simulink library "SHCLib"  (R2023a)
settings: Solver=VariableStepAuto  StartTime=0.0  StopTime=10.0  RelTol=1e-3
settings Model: Creator=hwx20  LastModifiedBy=hwx20

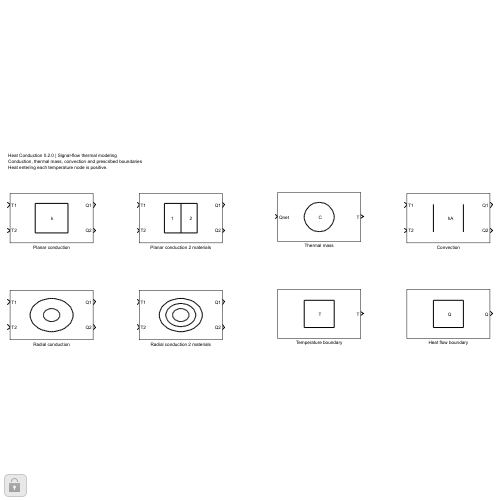
[thumbnail: Simulink's stored preview of the top-level diagram]
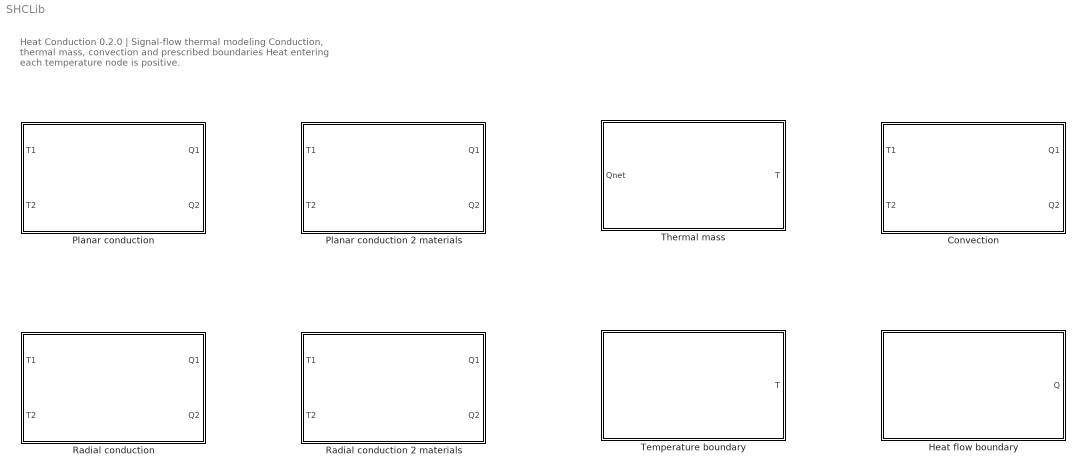
== system SHCLib ==
  note: Heat Conduction 0.2.0 | Signal-flow thermal modeling
      | Conduction, thermal mass, convection and prescribed boundaries
      | Heat entering each temperature node is positive.
  Convection : Subsystem  mask(SHC Convection){h=10, area=0.5}
      mask prompts: h "Heat transfer coefficient / 对流换热系数 [W/(m^2 K)]"; area "Heat transfer area / 换热面积 [m^2]"
      mask help:
      | Constant-coefficient convection / 常系数对流换热.
      | Inputs T1,T2 [same temperature scale]; outputs Q1,Q2 [W].
      | Q1=h*area*(T2-T1), Q2=-Q1. Positive heat enters the corresponding node.
      | h=0 gives zero heat flow. This element has no thermal storage.
      | It does not calculate fluid flow or infer h from flow conditions.
      mask init:
      | validateattributes(area,{'numeric'},{'real','scalar','finite','positive'},'SHC','area');
      | validateattributes(h,{'numeric'},{'real','scalar','finite','nonnegative'},'SHC','h');
      | validateattributes(h*area,{'numeric'},{'real','scalar','finite','nonnegative'},'SHC','convective conductance');
      mask Help: disp(get_param(gcb,'MaskDescription'));
      mask Display:
      | plot([.32 .32],[.22 .78]);
      | plot([.68 .68],[.22 .78]);
      | text(.5,.5,'hA');
      | port_label('input',1,'T1');
      | port_label('input',2,'T2');
      | port_label('output',1,'Q1');
      | port_label('output',2,'Q2');
  Heat flow boundary : Subsystem  mask(SHC Heat flow boundary){power=100}
      mask prompts: power "Prescribed heat power / 规定热功率 [W]"
      mask help:
      | Constant prescribed heat power / 恒热功率边界.
      | Output Q [W]: positive adds heat; negative removes heat.
      | Add this signal to the receiving thermal mass net heat input.
      | This is total heat power, not area-specific heat flux [W/m^2].
      | Use a standard Simulink source for a time-dependent heat-power signal.
      mask init:
      | validateattributes(power,{'numeric'},{'real','scalar','finite'},'SHC','power');
      mask Help: disp(get_param(gcb,'MaskDescription'));
      mask Display:
      | plot([.32 .32 .68 .68 .32],[.22 .78 .78 .22 .22]);
      | text(.5,.5,'Q');
      | port_label('output',1,'Q');
  Planar conduction : Subsystem  mask(SHC Planar conduction){lambda=10, distance=0.01, area=0.02}
      mask prompts: lambda "Thermal conductivity / 导热系数 [W/(m K)]"; distance "Distance between temperature nodes / 节点间距离 [m]"; area "Heat transfer area / 传热面积 [m^2]"
      mask help:
      | Single-material planar conduction.
      | R=distance/(lambda*area).
      | T1/T2: temperature [degC or K, use the same scale].
      | Q1/Q2: heat entering node 1/node 2 [W].
      | Q1=(T2-T1)/R; Q2=-Q1.
      | This is a resistance element. Add external thermal capacitances for storage.
      mask init:
      | validateattributes(lambda,{'numeric'},{'real','scalar','finite','positive'},'SHC','lambda');
      | validateattributes(distance,{'numeric'},{'real','scalar','finite','positive'},'SHC','distance');
      | validateattributes(area,{'numeric'},{'real','scalar','finite','positive'},'SHC','area');
      | 
      | validateattributes(distance/(lambda*area),{'numeric'},{'real','scalar','finite','positive'},'SHC','R_total');
      mask Help: disp(get_param(gcb,'MaskDescription'));
      mask Display:
      | plot([.30 .30 .70 .70 .30],[.20 .80 .80 .20 .20]);
      | text(.50,.50,'k');
      | port_label('input',1,'T1');
      | port_label('input',2,'T2');
      | port_label('output',1,'Q1');
      | port_label('output',2,'Q2');
  Planar conduction 2 materials : Subsystem  mask(SHC Planar conduction 2 materials){lambda1=1, distance1=0.005, lambda2=2, distance2=0.002, area=0.01, ctr=0.2}
      mask prompts: lambda1 "Material 1 conductivity / 材料1导热系数 [W/(m K)]"; distance1 "Node 1 to interface / 节点1到界面距离 [m]"; lambda2 "Material 2 conductivity / 材料2导热系数 [W/(m K)]"; distance2 "Interface to node 2 / 界面到节点2距离 [m]"; area "Heat transfer area / 传热面积 [m^2]"; ctr "Total contact resistance / 界面总热阻 [K/W]"
      mask help:
      | Two planar material layers in series, with optional contact resistance.
      | R=distance1/(lambda1*area)+distance2/(lambda2*area)+ctr.
      | ctr is TOTAL resistance [K/W], not area-specific resistance.
      | T1/T2: temperature [degC or K, use the same scale].
      | Q1/Q2: heat entering node 1/node 2 [W].
      | Q1=(T2-T1)/R; Q2=-Q1.
      | This is a resistance element. Add external thermal capacitances for storage.
      mask init:
      | validateattributes(lambda1,{'numeric'},{'real','scalar','finite','positive'},'SHC','lambda1');
      | validateattributes(lambda2,{'numeric'},{'real','scalar','finite','positive'},'SHC','lambda2');
      | validateattributes(area,{'numeric'},{'real','scalar','finite','positive'},'SHC','area');
      | validateattributes(distance1,{'numeric'},{'real','scalar','finite','nonnegative'},'SHC','distance1');
      | validateattributes(distance2,{'numeric'},{'real','scalar','finite','nonnegative'},'SHC','distance2');
      | validateattributes(ctr,{'numeric'},{'real','scalar','finite','nonnegative'},'SHC','ctr');
      | 
      | validateattributes(distance1/(lambda1*area)+distance2/(lambda2*area)+ctr,{'numeric'},{'real','scalar','finite','positive'},'SHC','R_total');
      mask Help: disp(get_param(gcb,'MaskDescription'));
      mask Display:
      | plot([.30 .30 .70 .70 .30],[.20 .80 .80 .20 .20]);
      | plot([.50 .50],[.20 .80]);
      | text(.39,.50,'1');text(.61,.50,'2');
      | port_label('input',1,'T1');
      | port_label('input',2,'T2');
      | port_label('output',1,'Q1');
      | port_label('output',2,'Q2');
  Radial conduction : Subsystem  mask(SHC Radial conduction){lambda=15, le=0.1, diamInt=0.02, diamExt=0.04}
      mask prompts: lambda "Thermal conductivity / 导热系数 [W/(m K)]"; le "Axial length / 轴向长度 [m]"; diamInt "Inner temperature-node diameter / 内侧节点直径 [m]"; diamExt "Outer temperature-node diameter / 外侧节点直径 [m]"
      mask help:
      | One cylindrical shell, radial conduction. T1 is inside; T2 is outside.
      | R=log(diamExt/diamInt)/(2*pi*lambda*le).
      | The inner diameter must be positive.
      | T1/T2: temperature [degC or K, use the same scale].
      | Q1/Q2: heat entering node 1/node 2 [W].
      | Q1=(T2-T1)/R; Q2=-Q1.
      | This is a resistance element. Add external thermal capacitances for storage.
      mask init:
      | validateattributes(lambda,{'numeric'},{'real','scalar','finite','positive'},'SHC','lambda');
      | validateattributes(le,{'numeric'},{'real','scalar','finite','positive'},'SHC','le');
      | validateattributes(diamInt,{'numeric'},{'real','scalar','finite','positive'},'SHC','diamInt');
      | validateattributes(diamExt,{'numeric'},{'real','scalar','finite','positive'},'SHC','diamExt');
      | assert(diamExt>diamInt, 'SHC:InvalidGeometry', 'Require 0 < diamInt < diamExt.');
      | validateattributes(log(diamExt/diamInt)/(2*pi*lambda*le),{'numeric'},{'real','scalar','finite','positive'},'SHC','R_total');
      mask Help: disp(get_param(gcb,'MaskDescription'));
      mask Display:
      | plot(.5+.26*cos(0:pi/32:2*pi),.5+.34*sin(0:pi/32:2*pi));
      | plot(.5+.10*cos(0:pi/32:2*pi),.5+.13*sin(0:pi/32:2*pi));
      | port_label('input',1,'T1');
      | port_label('input',2,'T2');
      | port_label('output',1,'Q1');
      | port_label('output',2,'Q2');
  Radial conduction 2 materials : Subsystem  mask(SHC Radial conduction 2 materials){lambda1=15, lambda2=0.2, le=0.1, diamInt=0.02, diamCt=0.024, diamExt=0.04, ctr=0.05}
      mask prompts: lambda1 "Inner material conductivity / 内层导热系数 [W/(m K)]"; lambda2 "Outer material conductivity / 外层导热系数 [W/(m K)]"; le "Axial length / 轴向长度 [m]"; diamInt "Inner temperature-node diameter / 内侧节点直径 [m]"; diamCt "Material interface diameter / 材料界面直径 [m]"; diamExt "Outer temperature-node diameter / 外侧节点直径 [m]"; ctr "Total contact resistance / 界面总热阻 [K/W]"
      mask help:
      | Two coaxial cylindrical shells in series. T1 is inside; T2 is outside.
      | R=log(diamCt/diamInt)/(2*pi*lambda1*le)+log(diamExt/diamCt)/(2*pi*lambda2*le)+ctr.
      | ctr is TOTAL resistance [K/W], not area-specific resistance.
      | T1/T2: temperature [degC or K, use the same scale].
      | Q1/Q2: heat entering node 1/node 2 [W].
      | Q1=(T2-T1)/R; Q2=-Q1.
      | This is a resistance element. Add external thermal capacitances for storage.
      mask init:
      | validateattributes(lambda1,{'numeric'},{'real','scalar','finite','positive'},'SHC','lambda1');
      | validateattributes(lambda2,{'numeric'},{'real','scalar','finite','positive'},'SHC','lambda2');
      | validateattributes(le,{'numeric'},{'real','scalar','finite','positive'},'SHC','le');
      | validateattributes(diamInt,{'numeric'},{'real','scalar','finite','positive'},'SHC','diamInt');
      | validateattributes(diamCt,{'numeric'},{'real','scalar','finite','positive'},'SHC','diamCt');
      | validateattributes(diamExt,{'numeric'},{'real','scalar','finite','positive'},'SHC','diamExt');
      | validateattributes(ctr,{'numeric'},{'real','scalar','finite','nonnegative'},'SHC','ctr');
      | assert(diamInt<diamCt && diamCt<diamExt, 'SHC:InvalidGeometry', 'Require 0 < diamInt < diamCt < diamExt.');
      | validateattributes(log(diamCt/diamInt)/(2*pi*lambda1*le)+log(diamExt/diamCt)/(2*pi*lambda2*le)+ctr,{'numeric'},{'real','scalar','finite','positive'},'SHC','R_total');
      mask Help: disp(get_param(gcb,'MaskDescription'));
      mask Display:
      | plot(.5+.26*cos(0:pi/32:2*pi),.5+.34*sin(0:pi/32:2*pi));
      | plot(.5+.10*cos(0:pi/32:2*pi),.5+.13*sin(0:pi/32:2*pi));
      | plot(.5+.18*cos(0:pi/32:2*pi),.5+.235*sin(0:pi/32:2*pi));
      | port_label('input',1,'T1');
      | port_label('input',2,'T2');
      | port_label('output',1,'Q1');
      | port_label('output',2,'Q2');
  Temperature boundary : Subsystem  mask(SHC Temperature boundary){temperature=20}
      mask prompts: temperature "Prescribed temperature / 规定温度 [degC or K]"
      mask help:
      | Constant prescribed temperature / 恒温边界.
      | Output T is a scalar Simulink temperature signal. No heat-flow input.
      | Connect to one side of a conduction/convection element.
      | The boundary represents an ideal reservoir; its temperature is not integrated.
      | A time-dependent boundary can instead use any compatible Simulink source.
      mask init:
      | validateattributes(temperature,{'numeric'},{'real','scalar','finite'},'SHC','temperature');
      mask Help: disp(get_param(gcb,'MaskDescription'));
      mask Display:
      | plot([.32 .32 .68 .68 .32],[.22 .78 .78 .22 .22]);
      | text(.5,.5,'T');
      | port_label('output',1,'T');
  Thermal mass : Subsystem  mask(SHC Thermal mass){mass=1, cp=1000, Tinit=20}
      mask prompts: mass "Mass / 质量 [kg]"; cp "Specific heat / 比热容 [J/(kg K)]"; Tinit "Initial temperature / 初始温度 [degC or K]"
      mask help:
      | Constant thermal capacitance / 常热容节点.
      | Input Qnet [W]: positive into this body. Output T [degC or K].
      | dT/dt=Qnet/(mass*cp), T(0)=Tinit. Sum all incoming heat flows first.
      | Uses a continuous Integrator: select a continuous solver (e.g. ode4 or ode45).
      | No ambient loss or heat generation is included internally.
      mask init:
      | validateattributes(mass,{'numeric'},{'real','scalar','finite','positive'},'SHC','mass');
      | validateattributes(cp,{'numeric'},{'real','scalar','finite','positive'},'SHC','cp');
      | validateattributes(Tinit,{'numeric'},{'real','scalar','finite'},'SHC','Tinit');
      | validateattributes(mass*cp,{'numeric'},{'real','scalar','finite','positive'},'SHC','thermal capacitance');
      mask Help: disp(get_param(gcb,'MaskDescription'));
      mask Display:
      | plot(.5+.18*cos(0:pi/32:2*pi),.5+.30*sin(0:pi/32:2*pi));
      | text(.5,.5,'C');
      | port_label('input',1,'Qnet');
      | port_label('output',1,'T');

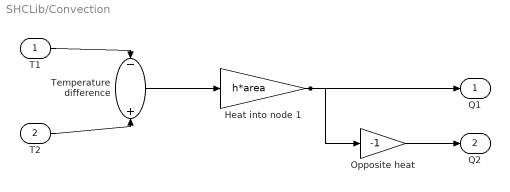
== system SHCLib/Convection ==
  T1 : Inport  PortDimensions=1
  T2 : Inport  Port=2  PortDimensions=1
  Heat into node 1 : Gain  Gain=h*area
  Opposite heat : Gain  Gain=-1
  Temperature difference : Sum  Inputs=-+
  Q1 : Outport
  Q2 : Outport  Port=2
  wires:
  T1/1 -> Temperature difference/1
  T2/1 -> Temperature difference/2
  Temperature difference/1 -> Heat into node 1/1
  Heat into node 1/1 -> Q1/1, Opposite heat/1
  Opposite heat/1 -> Q2/1

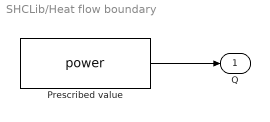
== system SHCLib/Heat flow boundary ==
  Prescribed value : Constant  Value=power
  Q : Outport
  wires:
  Prescribed value/1 -> Q/1

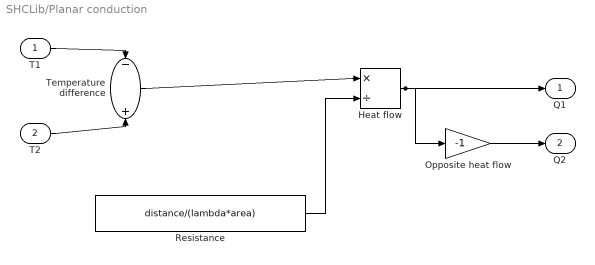
== system SHCLib/Planar conduction ==
  T1 : Inport
  T2 : Inport  Port=2
  Heat flow : Product  Inputs=*/
  Opposite heat flow : Gain  Gain=-1
  Resistance : Constant  Value=distance/(lambda*area)
  Temperature difference : Sum  Inputs=-+
  Q1 : Outport
  Q2 : Outport  Port=2
  wires:
  T1/1 -> Temperature difference/1
  T2/1 -> Temperature difference/2
  Temperature difference/1 -> Heat flow/1
  Resistance/1 -> Heat flow/2
  Heat flow/1 -> Q1/1, Opposite heat flow/1
  Opposite heat flow/1 -> Q2/1

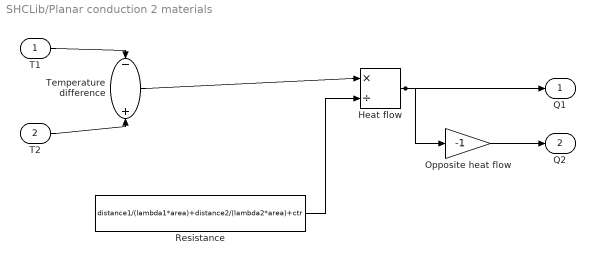
== system SHCLib/Planar conduction 2 materials ==
  T1 : Inport
  T2 : Inport  Port=2
  Heat flow : Product  Inputs=*/
  Opposite heat flow : Gain  Gain=-1
  Resistance : Constant  Value=distance1/(lambda1*area)+distance2/(lambda2*area)+ctr
  Temperature difference : Sum  Inputs=-+
  Q1 : Outport
  Q2 : Outport  Port=2
  wires:
  T1/1 -> Temperature difference/1
  T2/1 -> Temperature difference/2
  Temperature difference/1 -> Heat flow/1
  Resistance/1 -> Heat flow/2
  Heat flow/1 -> Q1/1, Opposite heat flow/1
  Opposite heat flow/1 -> Q2/1

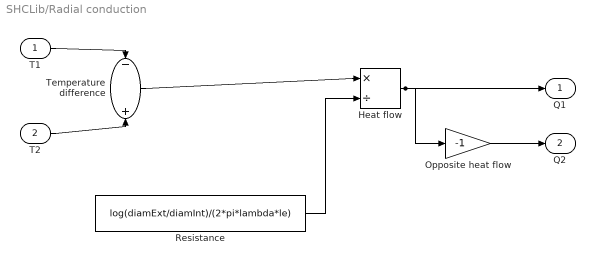
== system SHCLib/Radial conduction ==
  T1 : Inport
  T2 : Inport  Port=2
  Heat flow : Product  Inputs=*/
  Opposite heat flow : Gain  Gain=-1
  Resistance : Constant  Value=log(diamExt/diamInt)/(2*pi*lambda*le)
  Temperature difference : Sum  Inputs=-+
  Q1 : Outport
  Q2 : Outport  Port=2
  wires:
  T1/1 -> Temperature difference/1
  T2/1 -> Temperature difference/2
  Temperature difference/1 -> Heat flow/1
  Resistance/1 -> Heat flow/2
  Heat flow/1 -> Q1/1, Opposite heat flow/1
  Opposite heat flow/1 -> Q2/1

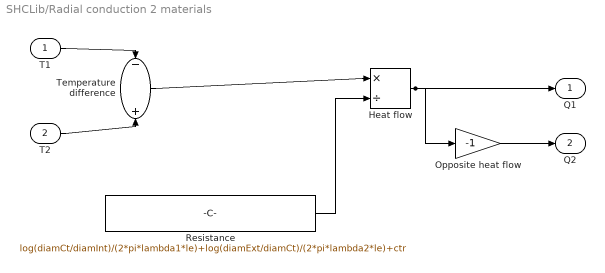
== system SHCLib/Radial conduction 2 materials ==
  T1 : Inport
  T2 : Inport  Port=2
  Heat flow : Product  Inputs=*/
  Opposite heat flow : Gain  Gain=-1
  Resistance : Constant  Value=log(diamCt/diamInt)/(2*pi*lambda1*le)+log(diamExt/diamCt)/(2*pi*lambda2*le)+ctr
  Temperature difference : Sum  Inputs=-+
  Q1 : Outport
  Q2 : Outport  Port=2
  wires:
  T1/1 -> Temperature difference/1
  T2/1 -> Temperature difference/2
  Temperature difference/1 -> Heat flow/1
  Resistance/1 -> Heat flow/2
  Heat flow/1 -> Q1/1, Opposite heat flow/1
  Opposite heat flow/1 -> Q2/1

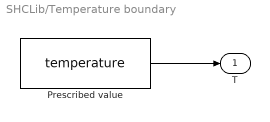
== system SHCLib/Temperature boundary ==
  Prescribed value : Constant  Value=temperature
  T : Outport
  wires:
  Prescribed value/1 -> T/1

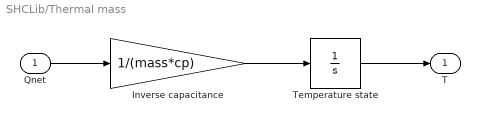
== system SHCLib/Thermal mass ==
  Qnet : Inport  PortDimensions=1
  Inverse capacitance : Gain  Gain=1/(mass*cp)
  Temperature state : Integrator  InitialCondition=Tinit
  T : Outport
  wires:
  Qnet/1 -> Inverse capacitance/1
  Inverse capacitance/1 -> Temperature state/1
  Temperature state/1 -> T/1
